simulink model "DSSS"  (R2018b)
settings: Solver=VariableStepAuto  StartTime=0.0  StopTime=10.0  RelTol=1e-3
libraries: commdigbbndpm3 x2, commseqgen3 x2, commchan3 x1, commsink2 x1, simulink x1, commfilt2 x1, commrandsrc3 x1
settings Model: Creator=asus  LastModifiedBy=asus

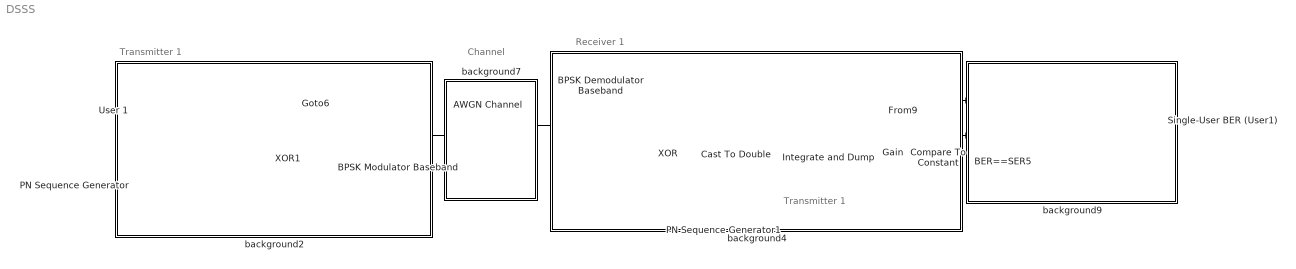
== system DSSS ==
  note: Receiver 1
  note: Channel
  note: Transmitter 1
  note: Transmitter 1
  AWGN Channel : commchan3/AWGN Channel  InputProcessing=Columns as channels (frame based)  seed=1237  noiseMode="Signal to noise ratio  (SNR)"  EbNodB=10  EsNodB=25  SNRdB=-4  bitsPerSym=1  Ps=1/2  Tsym=ts  variance=1
  BER==SER5 : commsink2/Error Rate Calculation  N=0  st_delay=0  cp_mode=Entire frame  subframe=[]  PMode=Port  WsName=ErrorVec  RsMode2=off  stop=off  numErr=100  maxBits=1e6
  BPSK Demodulator Baseband : commdigbbndpm3/BPSK Demodulator Baseband  DecType=Hard decision  VarSource=Dialog  Variance=1  Ph=0  outDtype=Inherit via internal rule  derotateFactorWordLen=16  derotateFactorDataTypeStr=Inherit: Same word length as input  derotateFactorLastDataTypeStr=Inherit: Same word length as input
  BPSK Modulator Baseband : commdigbbndpm3/BPSK Modulator Baseband  Ph=0  outDtype=double  outWordLen=16  outUDDataType=sfix(16)  outFracLenMode=Best precision  outFracLen=15  outDataTypeStr=double  outLastDataTypeStr=double
  Cast To Double : DataTypeConversion  OutDataTypeStr=double
  Compare To Constant : simulink/Logic and Bit Operations/Compare To Constant  relop=>=  const=0.5  OutDataTypeStr=boolean
  Gain : Gain  Gain=1/7  OutMin=[0]  OutMax=[1]
  Integrate and Dump : commfilt2/Integrate and Dump  obssamples=7  offsetsamples=0  nodump=off  roundingMode=Floor  overflowMode=off  outputDataTypeStr=Inherit: Same as accumulator  outputLastDataTypeStr=Inherit: Same as accumulator
  PN Sequence Generator : commseqgen3/PN Sequence Generator  poly='z^3 + z + 1'  ini_sta=[0 0 1]  outBitMaskSource=Dialog parameter  shift=0  outVarSiz=off  maxOutSizeMode=Dialog parameter  maxOutSize=[10 1]  Ts=1/7*1000  sampPerFrame=7  reset=off  bitPackedOutputs=off  outDataType=double  numPackedBits=8  bitPackDataSigned=off  bitPackedOutDType=double
      settings: SourceProductName=Communications System Toolbox
  PN Sequence Generator1 : commseqgen3/PN Sequence Generator  poly='z^3+ z + 1'  ini_sta=[0 0 1]  outBitMaskSource=Dialog parameter  shift=0  outVarSiz=off  maxOutSizeMode=Dialog parameter  maxOutSize=[10 1]  Ts=1/7*1000  sampPerFrame=7  reset=off  bitPackedOutputs=off  outDataType=double  numPackedBits=8  bitPackDataSigned=off  bitPackedOutDType=double
      settings: SourceProductName=Communications System Toolbox
  Single-User BER (User1) : Display
  User 1 : commrandsrc3/Random Integer Generator  SetSize=2  SeedSource=Parameter  Seed=37  SampleTime=1/1000  SamplesPerFrame=1  OutputDataType=boolean  SimulateUsing=Interpreted execution
  XOR : Logic  Operator=XOR  IconShape=distinctive  AllPortsSameDT=off  OutDataTypeStr=boolean
  XOR1 : Logic  Operator=XOR  IconShape=distinctive  AllPortsSameDT=off  OutDataTypeStr=boolean
  background2 : Subsystem
      mask Display: disp('')
  background4 : Subsystem
      mask Display: disp('')
  background7 : Subsystem
      mask Display: disp('')
  background9 : Subsystem
      mask Display: disp('')
  tag scope: User1Tx=global
  wires:
  User 1/1 -> XOR1/1, [User1Tx]
  BPSK Modulator Baseband/1 -> AWGN Channel/1
  XOR/1 -> Cast To Double/1
  PN Sequence Generator/1 -> XOR1/2
  XOR1/1 -> BPSK Modulator Baseband/1
  BPSK Demodulator Baseband/1 -> XOR/1
  [User1Tx] -> BER==SER5/1
  Cast To Double/1 -> Integrate and Dump/1
  BER==SER5/1 -> Single-User BER (User1)/1
  Integrate and Dump/1 -> Gain/1
  PN Sequence Generator1/1 -> XOR/2
  AWGN Channel/1 -> BPSK Demodulator Baseband/1
  Gain/1 -> Compare To Constant/1
  Compare To Constant/1 -> BER==SER5/2

== system DSSS/background2 ==

== system DSSS/background4 ==

== system DSSS/background7 ==

== system DSSS/background9 ==
